simulink model "Copy_of_single_camera_q_dot"  (R2025b)
settings: Solver=FixedStepDiscrete  StartTime=0  StopTime=inf  FixedStep=Ts  RelTol=1e-3
InitFcn:
  | % 获取当前.slx模型所在文件夹
  | model_path = fileparts(which(gcs));
  | % 向上跳转、拼接目标函数所在文件夹（根据你的目录调整）
  | func_folder = fullfile(model_path,'..', 'config');
  | % 添加到搜索路径
  | addpath(func_folder);
  | % 执行初始化函数
  | init_single_camera_q_dot_tracking;
undefined symbols (not defined in the file or in its folder): camera_velocity_feedback_timeout_sec, controller_enable, cx, cy, data, data_SL_Info, depth_safe_max, depth_safe_min, depth_safety_gain, ekf_gate_threshold, enable_ekf_feedforward, enable_proportional, fx, fy, joint_acceleration_limit, joint_nominal_configuration, joint_position_max, joint_position_min, joint_soft_margin, joint_state_timeout_sec, joint_velocity_limit, k_ff, Kpx, Kpy, measurement_reset_timeout, nullspace_posture_gain, P0, Q_ekf, R_ekf, required_valid_frames, singularity_sigma_stop, singularity_sigma_warn, target_timeout_sec, task_velocity_filter_tau, Ts, visual_damping_max, visual_damping_min, visual_min_depth, Z_hat
libraries: ros2lib x4, robotmaniplib x2
(part 1 of 2)
Description:
  | Fixed-focus monocular XY target tracking. Outputs camera-frame [vx vy 0 0 0 0]; robot kinematics remain external.
settings Model: Creator=ASUS  LastModifiedBy=harry
settings DataIOCC: SignalLogging=off

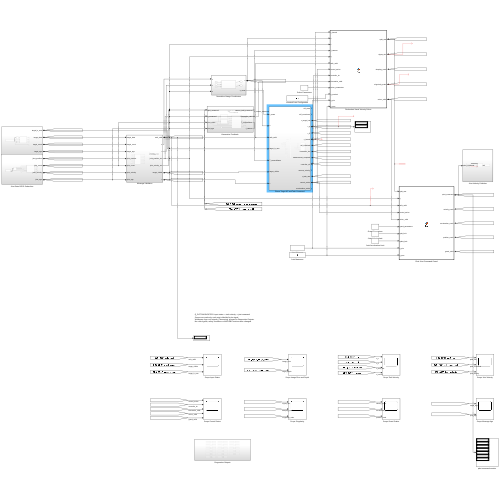
[thumbnail: Simulink's stored preview of the top-level diagram]
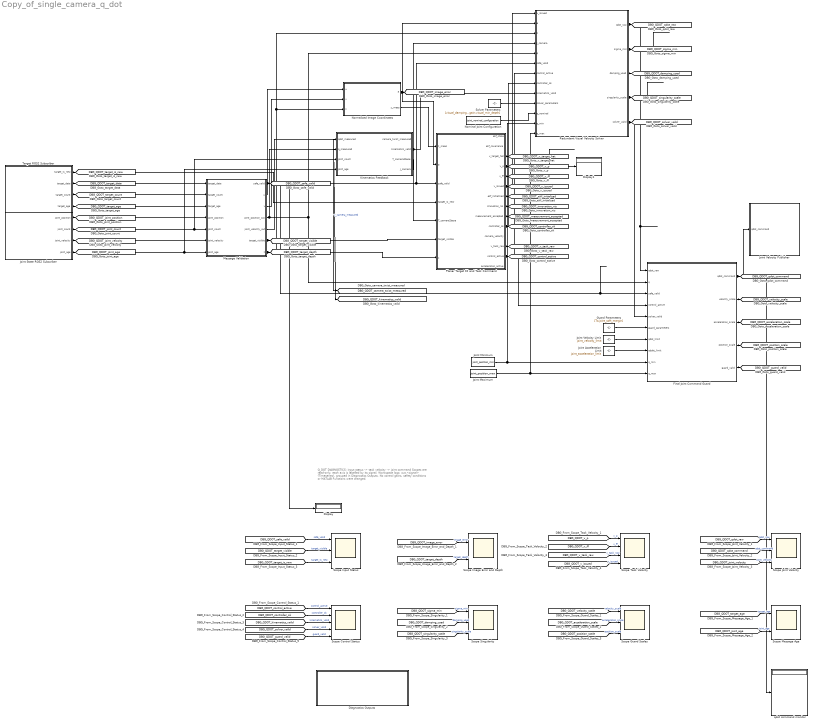
== system Copy_of_single_camera_q_dot ==
  note: Q_DOT DIAGNOSTICS: input status -> task velocity -> joint command
      | Scopes are read-only; each axis is labelled by its signal.
      | Workspace logs: out.<signal> (Timeseries), grouped in Diagnostics Outputs.
      | No control gains, safety conditions or MATLAB Functions were changed.
  Diagnostics Outputs : Subsystem
  Display : Display
  Display1 : Display
  Final Joint Command Guard : MATLAB Function  TreatAsAtomicUnit=on
  Guard Parameters : Constant  Value=[Ts;joint_soft_margin]
  Joint Acceleration Limit : Constant  Value=joint_acceleration_limit
  Joint Maximum : Constant  Value=joint_position_max
  Joint Minimum : Constant  Value=joint_position_min
  Joint State ROS2 Subscriber : Subsystem
  Joint Velocity Limit : Constant  Value=joint_velocity_limit
  Joint Velocity Publisher : Subsystem
  Kinematics Feedback : Subsystem
  Message Validation : Subsystem
  Nominal Joint Configuration : Constant  Value=joint_nominal_configuration
  Normalized Image Coordinates : Subsystem
  Planar Target KF and Task Command : Subsystem
  Redundant Visual Velocity Solver : MATLAB Function  TreatAsAtomicUnit=on
  Scope Control Status : Scope  NumInputPorts=5
      settings: TimeSpan=10  ActiveDisplayString=5  Title=guard_valid  ActiveDisplayYMinimum=-0.037001953201183713  ActiveDisplayYMaximum=0.0101088347899616  DataLoggingVariableName=ScopeData4
  Scope Guard Scales : Scope  NumInputPorts=3
      settings: TimeSpan=10  ActiveDisplayString=3  Title=position_scale  ActiveDisplayYMinimum=-12.068513318672558  ActiveDisplayYMaximum=6.6876450330275015  DataLoggingVariableName=ScopeData6
  Scope Image Error and Depth : Scope  NumInputPorts=2
      settings: TimeSpan=10  Title=target_depth  ActiveDisplayYMinimum=-1  ActiveDisplayYMaximum=1
  Scope Input Status : Scope  NumInputPorts=3
      settings: TimeSpan=10  ActiveDisplayString=3  Title=target_is_new  ActiveDisplayYMinimum=-1.6084422447956979  ActiveDisplayYMaximum=1.406793571934575  DataLoggingVariableName=ScopeData7
  Scope Joint Velocity : Scope  NumInputPorts=3
      settings: TimeSpan=10  ActiveDisplayString=3  Title=joint_velocity  ActiveDisplayYMinimum=-1.0517167509781138  ActiveDisplayYMaximum=1.0307773782957734  DataLoggingVariableName=ScopeData2
  Scope Message Age : Scope  NumInputPorts=2
      settings: TimeSpan=10  Title=joint_age  ActiveDisplayYMinimum=-1  ActiveDisplayYMaximum=1
  Scope Singularity : Scope  NumInputPorts=3
      settings: TimeSpan=10  ActiveDisplayString=3  Title=singularity_scale  ActiveDisplayYMinimum=-3.3735923675324466  ActiveDisplayYMaximum=2.902388236211491  DataLoggingVariableName=ScopeData5
  Scope Task Velocity : Scope  NumInputPorts=4
      settings: TimeSpan=10  ActiveDisplayString=4  Title=v_issued  ActiveDisplayYMinimum=-1  ActiveDisplayYMaximum=1  DataLoggingVariableName=ScopeData3
  Solver Parameters : Constant  Value=[visual_damping_min;visual_damping_max;singularity_sigma_stop;singularity_sigma_warn;nullspace_posture_gain;depth_safe_min;depth_safe_max;depth_safety_gain;visual_min_depth]
  Target ROS2 Subscriber : Subsystem
  qdot command monitor : Display
  tag scope: DBG_QDOT_acceleration_scale=global, DBG_QDOT_camera_twist_measured=global, DBG_QDOT_control_active=global, DBG_QDOT_controller_ok=global, DBG_QDOT_damping_used=global, DBG_QDOT_ekf_initialized=global, DBG_QDOT_guard_valid=global, DBG_QDOT_image_error=global, DBG_QDOT_innovation_nis=global, DBG_QDOT_joint_age=global, DBG_QDOT_joint_count=global, DBG_QDOT_joint_position=global, DBG_QDOT_joint_velocity=global, DBG_QDOT_kinematics_valid=global, DBG_QDOT_measurement_accepted=global, DBG_QDOT_position_scale=global, DBG_QDOT_qdot_command=global, DBG_QDOT_qdot_raw=global, DBG_QDOT_safe_valid=global, DBG_QDOT_sigma_min=global, DBG_QDOT_singularity_scale=global, DBG_QDOT_solver_valid=global, DBG_QDOT_target_age=global, DBG_QDOT_target_count=global, DBG_QDOT_target_data=global, DBG_QDOT_target_depth=global, DBG_QDOT_target_is_new=global, DBG_QDOT_target_visible=global, DBG_QDOT_v_ff=global, DBG_QDOT_v_issued=global, DBG_QDOT_v_p=global, DBG_QDOT_v_target_hat=global, DBG_QDOT_v_task_raw=global, DBG_QDOT_velocity_scale=global
  wires:
  Final Joint Command Guard/1(qdot_command) -> Joint Velocity Publisher/1(qdot_command), qdot command monitor/1, [DBG_QDOT_qdot_command]
  Message Validation/4(joint_position_out) -> Final Joint Command Guard/2(q), Redundant Visual Velocity Solver/5(q), Kinematics Feedback/2(q_measured)
  Kinematics Feedback/2(kinematics_valid) -> Redundant Visual Velocity Solver/9(kinematics_valid), [DBG_QDOT_kinematics_valid]
  Joint Velocity Limit/1 -> Final Joint Command Guard/7(qdot_limit)
  Message Validation/2(u) -> Normalized Image Coordinates/1(u)
  Target ROS2 Subscriber/3(target_count) -> Message Validation/2(target_count), [DBG_QDOT_target_count]
  Redundant Visual Velocity Solver/5(solver_valid) -> Final Joint Command Guard/5(solver_valid), [DBG_QDOT_solver_valid]
  Target ROS2 Subscriber/1(target_is_new) -> Planar Target KF and Task Command/4(target_is_new), [DBG_QDOT_target_is_new]
  Planar Target KF and Task Command/10(controller_ok) -> Redundant Visual Velocity Solver/8(controller_ok), [DBG_QDOT_controller_ok]
  Message Validation/5(joint_velocity_out) -> Kinematics Feedback/1(qdot_measured)
  Message Validation/7(z) -> Redundant Visual Velocity Solver/3(z), Normalized Image Coordinates/3(z), Planar Target KF and Task Command/7(z), [DBG_QDOT_target_depth]
  Joint Acceleration Limit/1 -> Final Joint Command Guard/8(qddot_limit)
  Joint State ROS2 Subscriber/4(joint_age) -> Kinematics Feedback/4(joint_age), Message Validation/7(joint_age), [DBG_QDOT_joint_age]
  Joint State ROS2 Subscriber/3(joint_velocity) -> Message Validation/6(joint_velocity), [DBG_QDOT_joint_velocity]
  Message Validation/6(target_visible) -> Planar Target KF and Task Command/6(target_visible), [DBG_QDOT_target_visible]
  Kinematics Feedback/4(J_camera) -> Redundant Visual Velocity Solver/4(J_camera)
  Redundant Visual Velocity Solver/1(qdot_raw) -> [DBG_QDOT_qdot_raw], Final Joint Command Guard/1(qdot_raw)
  Message Validation/1(safe_valid) -> Final Joint Command Guard/3(safe_valid), Redundant Visual Velocity Solver/6(safe_valid), Planar Target KF and Task Command/3(safe_valid), Display/1, [DBG_QDOT_safe_valid]
  Message Validation/3(v) -> Normalized Image Coordinates/2(v)
  Planar Target KF and Task Command/13(control_active) -> Redundant Visual Velocity Solver/7(control_active), Final Joint Command Guard/4(control_active), [DBG_QDOT_control_active]
  Joint State ROS2 Subscriber/1(joint_position) -> Message Validation/4(joint_position), [DBG_QDOT_joint_position]
  Guard Parameters/1 -> Final Joint Command Guard/6(guard_parameters)
  Joint State ROS2 Subscriber/2(joint_count) -> Kinematics Feedback/3(joint_count), Message Validation/5(joint_count), [DBG_QDOT_joint_count]
  Normalized Image Coordinates/1(e) -> Planar Target KF and Task Command/2(e), Redundant Visual Velocity Solver/2(e), [DBG_QDOT_image_error]
  Target ROS2 Subscriber/2(target_data) -> Message Validation/1(target_data), [DBG_QDOT_target_data]
  Normalized Image Coordinates/2(z_meas) -> Planar Target KF and Task Command/1(z_meas)
  Kinematics Feedback/3(T_camera2base) -> Planar Target KF and Task Command/5(T_camera2base)
  Solver Parameters/1 -> Redundant Visual Velocity Solver/10(solver_parameters)
  Nominal Joint Configuration/1 -> Redundant Visual Velocity Solver/11(q_nominal)
  Joint Minimum/1 -> Redundant Visual Velocity Solver/12(q_min), Final Joint Command Guard/9(q_min)
  Joint Maximum/1 -> Final Joint Command Guard/10(q_max), Redundant Visual Velocity Solver/13(q_max)
  Target ROS2 Subscriber/4(target_age) -> Message Validation/3(target_age), [DBG_QDOT_target_age]
  Planar Target KF and Task Command/4(v_p) -> Display1/1, [DBG_QDOT_v_p]
  Planar Target KF and Task Command/6(v_issued) -> Redundant Visual Velocity Solver/1(v_issued), [DBG_QDOT_v_issued]
  Redundant Visual Velocity Solver/2(sigma_min) -> [DBG_QDOT_sigma_min]
  Redundant Visual Velocity Solver/4(singularity_scale) -> [DBG_QDOT_singularity_scale]
  Kinematics Feedback/1(camera_twist_measured) -> [DBG_QDOT_camera_twist_measured]  "v_camera_measured"
  Planar Target KF and Task Command/3(v_target_hat) -> [DBG_QDOT_v_target_hat]
  Planar Target KF and Task Command/5(v_ff) -> [DBG_QDOT_v_ff]
  Planar Target KF and Task Command/7(ekf_initialized) -> [DBG_QDOT_ekf_initialized]
  Planar Target KF and Task Command/8(innovation_nis) -> [DBG_QDOT_innovation_nis]
  Planar Target KF and Task Command/9(measurement_accepted) -> [DBG_QDOT_measurement_accepted]
  Planar Target KF and Task Command/12(v_task_raw) -> [DBG_QDOT_v_task_raw]
  Redundant Visual Velocity Solver/3(damping_used) -> [DBG_QDOT_damping_used]
  Final Joint Command Guard/2(velocity_scale) -> [DBG_QDOT_velocity_scale]
  Final Joint Command Guard/3(acceleration_scale) -> [DBG_QDOT_acceleration_scale]
  Final Joint Command Guard/4(position_scale) -> [DBG_QDOT_position_scale]
  Final Joint Command Guard/5(guard_valid) -> [DBG_QDOT_guard_valid]
  [DBG_QDOT_safe_valid] -> Scope Input Status/1  "safe_valid"
  [DBG_QDOT_target_visible] -> Scope Input Status/2  "target_visible"
  [DBG_QDOT_target_is_new] -> Scope Input Status/3  "target_is_new"
  [DBG_QDOT_image_error] -> Scope Image Error and Depth/1  "image_error"
  [DBG_QDOT_target_depth] -> Scope Image Error and Depth/2  "target_depth"
  [DBG_QDOT_v_p] -> Scope Task Velocity/1  "v_p"
  [DBG_QDOT_v_ff] -> Scope Task Velocity/2  "v_ff"
  [DBG_QDOT_v_task_raw] -> Scope Task Velocity/3  "v_task_raw"
  [DBG_QDOT_v_issued] -> Scope Task Velocity/4  "v_issued"
  [DBG_QDOT_qdot_raw] -> Scope Joint Velocity/1  "qdot_raw"
  [DBG_QDOT_qdot_command] -> Scope Joint Velocity/2  "qdot_command"
  [DBG_QDOT_joint_velocity] -> Scope Joint Velocity/3  "joint_velocity"
  [DBG_QDOT_control_active] -> Scope Control Status/1  "control_active"
  [DBG_QDOT_controller_ok] -> Scope Control Status/2  "controller_ok"
  [DBG_QDOT_kinematics_valid] -> Scope Control Status/3  "kinematics_valid"
  [DBG_QDOT_solver_valid] -> Scope Control Status/4  "solver_valid"
  [DBG_QDOT_guard_valid] -> Scope Control Status/5  "guard_valid"
  [DBG_QDOT_sigma_min] -> Scope Singularity/1  "sigma_min"
  [DBG_QDOT_damping_used] -> Scope Singularity/2  "damping_used"
  [DBG_QDOT_singularity_scale] -> Scope Singularity/3  "singularity_scale"
  [DBG_QDOT_velocity_scale] -> Scope Guard Scales/1  "velocity_scale"
  [DBG_QDOT_acceleration_scale] -> Scope Guard Scales/2  "acceleration_scale"
  [DBG_QDOT_position_scale] -> Scope Guard Scales/3  "position_scale"
  [DBG_QDOT_target_age] -> Scope Message Age/1  "target_age"
  [DBG_QDOT_joint_age] -> Scope Message Age/2  "joint_age"

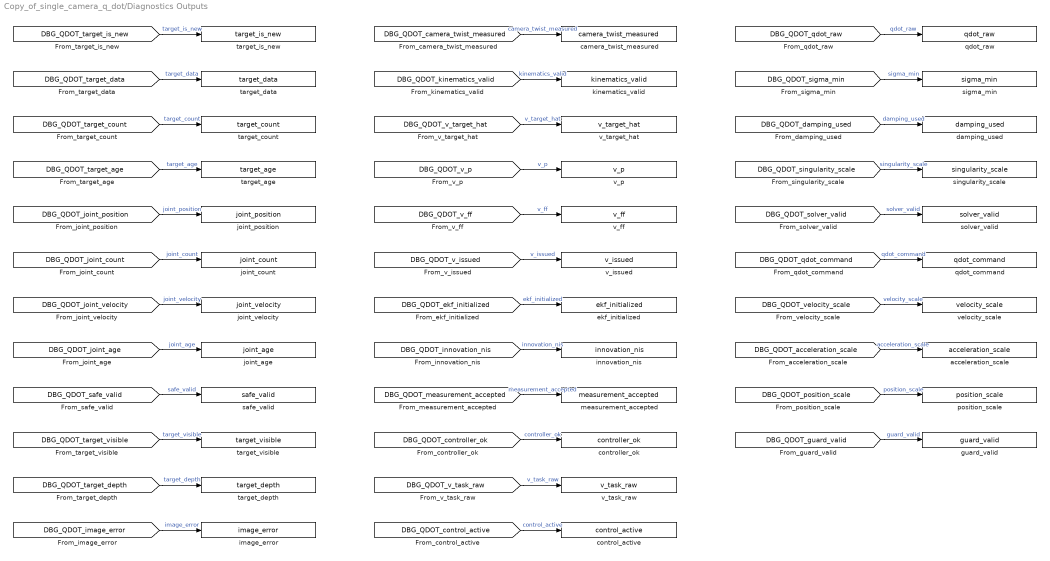
== system Copy_of_single_camera_q_dot/Diagnostics Outputs ==
  acceleration_scale : ToWorkspace  VariableName=acceleration_scale  SaveFormat=Timeseries  SampleTime=-1
  camera_twist_measured : ToWorkspace  VariableName=camera_twist_measured  SaveFormat=Timeseries  SampleTime=-1
  control_active : ToWorkspace  VariableName=control_active  SaveFormat=Timeseries  SampleTime=-1
  controller_ok : ToWorkspace  VariableName=controller_ok  SaveFormat=Timeseries  SampleTime=-1
  damping_used : ToWorkspace  VariableName=damping_used  SaveFormat=Timeseries  SampleTime=-1
  ekf_initialized : ToWorkspace  VariableName=ekf_initialized  SaveFormat=Timeseries  SampleTime=-1
  guard_valid : ToWorkspace  VariableName=guard_valid  SaveFormat=Timeseries  SampleTime=-1
  image_error : ToWorkspace  VariableName=image_error  SaveFormat=Timeseries  SampleTime=-1
  innovation_nis : ToWorkspace  VariableName=innovation_nis  SaveFormat=Timeseries  SampleTime=-1
  joint_age : ToWorkspace  VariableName=joint_age  SaveFormat=Timeseries  SampleTime=-1
  joint_count : ToWorkspace  VariableName=joint_count  SaveFormat=Timeseries  SampleTime=-1
  joint_position : ToWorkspace  VariableName=joint_position  SaveFormat=Timeseries  SampleTime=-1
  joint_velocity : ToWorkspace  VariableName=joint_velocity  SaveFormat=Timeseries  SampleTime=-1
  kinematics_valid : ToWorkspace  VariableName=kinematics_valid  SaveFormat=Timeseries  SampleTime=-1
  measurement_accepted : ToWorkspace  VariableName=measurement_accepted  SaveFormat=Timeseries  SampleTime=-1
  position_scale : ToWorkspace  VariableName=position_scale  SaveFormat=Timeseries  SampleTime=-1
  qdot_command : ToWorkspace  VariableName=qdot_command  SaveFormat=Timeseries  SampleTime=-1
  qdot_raw : ToWorkspace  VariableName=qdot_raw  SaveFormat=Timeseries  SampleTime=-1
  safe_valid : ToWorkspace  VariableName=safe_valid  SaveFormat=Timeseries  SampleTime=-1
  sigma_min : ToWorkspace  VariableName=sigma_min  SaveFormat=Timeseries  SampleTime=-1
  singularity_scale : ToWorkspace  VariableName=singularity_scale  SaveFormat=Timeseries  SampleTime=-1
  solver_valid : ToWorkspace  VariableName=solver_valid  SaveFormat=Timeseries  SampleTime=-1
  target_age : ToWorkspace  VariableName=target_age  SaveFormat=Timeseries  SampleTime=-1
  target_count : ToWorkspace  VariableName=target_count  SaveFormat=Timeseries  SampleTime=-1
  target_data : ToWorkspace  VariableName=target_data  SaveFormat=Timeseries  SampleTime=-1
  target_depth : ToWorkspace  VariableName=target_depth  SaveFormat=Timeseries  SampleTime=-1
  target_is_new : ToWorkspace  VariableName=target_is_new  SaveFormat=Timeseries  SampleTime=-1
  target_visible : ToWorkspace  VariableName=target_visible  SaveFormat=Timeseries  SampleTime=-1
  v_ff : ToWorkspace  VariableName=v_ff  SaveFormat=Timeseries  SampleTime=-1
  v_issued : ToWorkspace  VariableName=v_issued  SaveFormat=Timeseries  SampleTime=-1
  v_p : ToWorkspace  VariableName=v_p  SaveFormat=Timeseries  SampleTime=-1
  v_target_hat : ToWorkspace  VariableName=v_target_hat  SaveFormat=Timeseries  SampleTime=-1
  v_task_raw : ToWorkspace  VariableName=v_task_raw  SaveFormat=Timeseries  SampleTime=-1
  velocity_scale : ToWorkspace  VariableName=velocity_scale  SaveFormat=Timeseries  SampleTime=-1
  wires:
  [DBG_QDOT_target_is_new] -> target_is_new/1  "target_is_new"
  [DBG_QDOT_target_data] -> target_data/1  "target_data"
  [DBG_QDOT_target_count] -> target_count/1  "target_count"
  [DBG_QDOT_target_age] -> target_age/1  "target_age"
  [DBG_QDOT_joint_position] -> joint_position/1  "joint_position"
  [DBG_QDOT_joint_count] -> joint_count/1  "joint_count"
  [DBG_QDOT_joint_velocity] -> joint_velocity/1  "joint_velocity"
  [DBG_QDOT_joint_age] -> joint_age/1  "joint_age"
  [DBG_QDOT_safe_valid] -> safe_valid/1  "safe_valid"
  [DBG_QDOT_target_visible] -> target_visible/1  "target_visible"
  [DBG_QDOT_target_depth] -> target_depth/1  "target_depth"
  [DBG_QDOT_image_error] -> image_error/1  "image_error"
  [DBG_QDOT_camera_twist_measured] -> camera_twist_measured/1  "camera_twist_measured"
  [DBG_QDOT_kinematics_valid] -> kinematics_valid/1  "kinematics_valid"
  [DBG_QDOT_v_target_hat] -> v_target_hat/1  "v_target_hat"
  [DBG_QDOT_v_p] -> v_p/1  "v_p"
  [DBG_QDOT_v_ff] -> v_ff/1  "v_ff"
  [DBG_QDOT_v_issued] -> v_issued/1  "v_issued"
  [DBG_QDOT_ekf_initialized] -> ekf_initialized/1  "ekf_initialized"
  [DBG_QDOT_innovation_nis] -> innovation_nis/1  "innovation_nis"
  [DBG_QDOT_measurement_accepted] -> measurement_accepted/1  "measurement_accepted"
  [DBG_QDOT_controller_ok] -> controller_ok/1  "controller_ok"
  [DBG_QDOT_v_task_raw] -> v_task_raw/1  "v_task_raw"
  [DBG_QDOT_control_active] -> control_active/1  "control_active"
  [DBG_QDOT_qdot_raw] -> qdot_raw/1  "qdot_raw"
  [DBG_QDOT_sigma_min] -> sigma_min/1  "sigma_min"
  [DBG_QDOT_damping_used] -> damping_used/1  "damping_used"
  [DBG_QDOT_singularity_scale] -> singularity_scale/1  "singularity_scale"
  [DBG_QDOT_solver_valid] -> solver_valid/1  "solver_valid"
  [DBG_QDOT_qdot_command] -> qdot_command/1  "qdot_command"
  [DBG_QDOT_velocity_scale] -> velocity_scale/1  "velocity_scale"
  [DBG_QDOT_acceleration_scale] -> acceleration_scale/1  "acceleration_scale"
  [DBG_QDOT_position_scale] -> position_scale/1  "position_scale"
  [DBG_QDOT_guard_valid] -> guard_valid/1  "guard_valid"

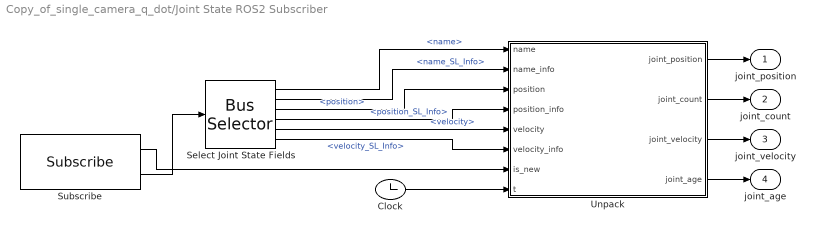
== system Copy_of_single_camera_q_dot/Joint State ROS2 Subscriber ==
  Clock : Clock
  Select Joint State Fields : BusSelector  OutputSignals=name,name_SL_Info,position,position_SL_Info,velocity,velocity_SL_Info
  Subscribe : ros2lib/Subscribe  topicSource=Select from ROS network  topic=/franka/joint_states  messageType=sensor_msgs/JointState  sampleTime=Ts  QOSHistory=Keep last  QOSDepth=1  QOSReliability=Best effort  QOSDurability=Volatile  QOSDeadline=Inf  QOSLifespan=Inf  QOSLiveliness=Automatic  QOSLeaseDuration=Inf  QOSAvoidROSNamespaceConventions=off
  Unpack : MATLAB Function  TreatAsAtomicUnit=on
  joint_position : Outport
  joint_count : Outport  Port=2
  joint_velocity : Outport  Port=3
  joint_age : Outport  Port=4
  wires:
  Unpack/1(joint_position) -> joint_position/1
  Unpack/2(joint_count) -> joint_count/1
  Unpack/3(joint_velocity) -> joint_velocity/1
  Unpack/4(joint_age) -> joint_age/1
  Subscribe/2 -> Select Joint State Fields/1
  Select Joint State Fields/1 -> Unpack/1(name)  "<name>"
  Select Joint State Fields/2 -> Unpack/2(name_info)  "<name_SL_Info>"
  Select Joint State Fields/3 -> Unpack/3(position)  "<position>"
  Select Joint State Fields/4 -> Unpack/4(position_info)  "<position_SL_Info>"
  Select Joint State Fields/5 -> Unpack/5(velocity)  "<velocity>"
  Select Joint State Fields/6 -> Unpack/6(velocity_info)  "<velocity_SL_Info>"
  Subscribe/1 -> Unpack/7(is_new)
  Clock/1 -> Unpack/8(t)

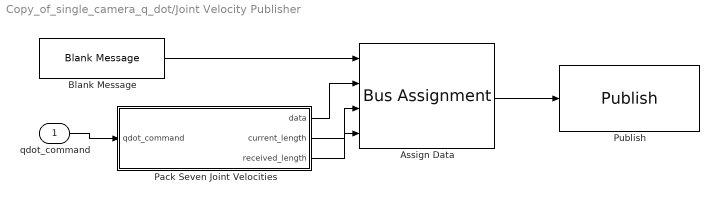
== system Copy_of_single_camera_q_dot/Joint Velocity Publisher ==
  qdot_command : Inport
  Assign Data : BusAssignment  AssignedSignals=data,data_SL_Info.CurrentLength,data_SL_Info.ReceivedLength
  Blank Message : ros2lib/Blank Message  messageClass=Message  entityType=std_msgs/Float64MultiArray  messageType=std_msgs/Float64MultiArray  SampleTime=Ts
  Pack Seven Joint Velocities : MATLAB Function  TreatAsAtomicUnit=on
  Publish : ros2lib/Publish  topicSource=Select from ROS network  topic=/joint_velocity_example_controller/commands  messageType=std_msgs/Float64MultiArray  QOSHistory=Keep last  QOSDepth=1  QOSReliability=Reliable  QOSDurability=Volatile  QOSDeadline=Inf  QOSLifespan=Inf  QOSLiveliness=Automatic  QOSLeaseDuration=Inf  QOSAvoidROSNamespaceConventions=off
  wires:
  ? -> ?
  qdot_command/1 -> Pack Seven Joint Velocities/1(qdot_command)
  Blank Message/1 -> Assign Data/1
  Pack Seven Joint Velocities/1(data) -> Assign Data/2
  Pack Seven Joint Velocities/2(current_length) -> Assign Data/3
  Pack Seven Joint Velocities/3(received_length) -> Assign Data/4
  Assign Data/1 -> Publish/1

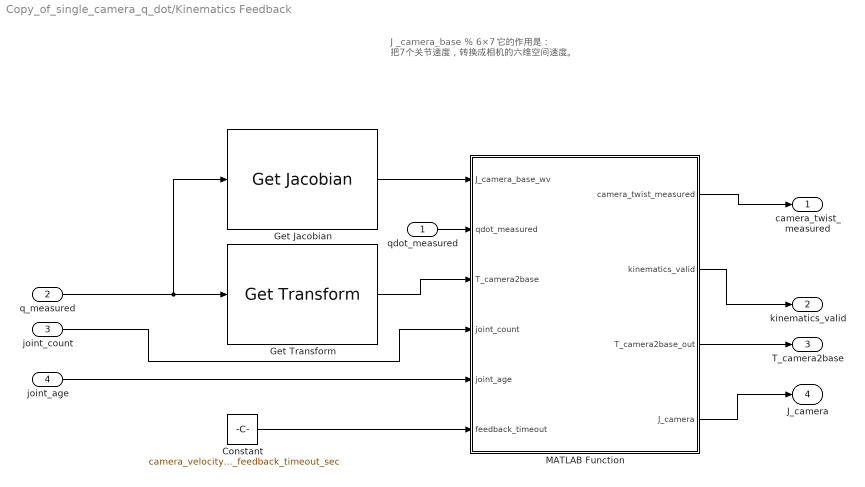
== system Copy_of_single_camera_q_dot/Kinematics Feedback ==
  note: J _camera_base % 6×7
      | 它的作用是：
      | 把7个关节速度，转换成相机的六维空间速度。
  qdot_measured : Inport
  q_measured : Inport  Port=2
  joint_count : Inport  Port=3
  joint_age : Inport  Port=4
  Constant : Constant  Value=camera_velocity_feedback_timeout_sec
  Get Jacobian : robotmaniplib/Get Jacobian  RigidBodyTree=fr3_camera_robot  EndEffector=camera_link  SimulateUsing=Interpreted execution
  Get Transform : robotmaniplib/Get Transform  RigidBodyTree=fr3_camera_robot  SourceBody=camera_link  TargetBody=base  SimulateUsing=Interpreted execution
  MATLAB Function : MATLAB Function  TreatAsAtomicUnit=on
  camera_twist_measured : Outport
  kinematics_valid : Outport  Port=2
  T_camera2base : Outport  Port=3
  J_camera : Outport  Port=4
  wires:
  q_measured/1 -> Get Jacobian/1, Get Transform/1
  qdot_measured/1 -> MATLAB Function/2(qdot_measured)
  Get Jacobian/1 -> MATLAB Function/1(J_camera_base_wv)
  Get Transform/1 -> MATLAB Function/3(T_camera2base)
  joint_count/1 -> MATLAB Function/4(joint_count)
  joint_age/1 -> MATLAB Function/5(joint_age)
  Constant/1 -> MATLAB Function/6(feedback_timeout)
  MATLAB Function/1(camera_twist_measured) -> camera_twist_measured/1
  MATLAB Function/2(kinematics_valid) -> kinematics_valid/1
  MATLAB Function/3(T_camera2base_out) -> T_camera2base/1
  MATLAB Function/4(J_camera) -> J_camera/1

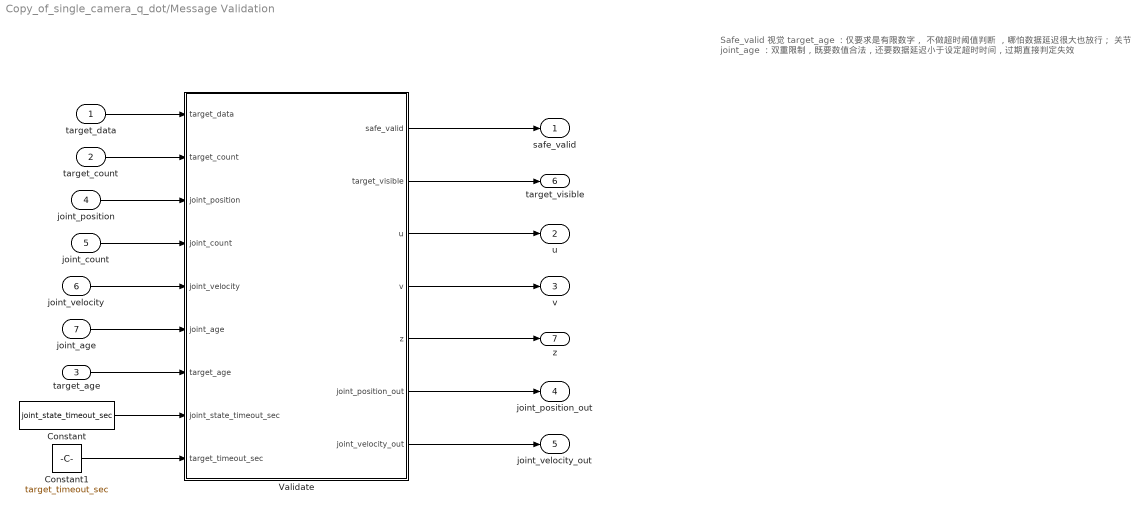
== system Copy_of_single_camera_q_dot/Message Validation ==
  note: Safe_valid
      | 视觉 target_age ：仅要求是有限数字， 不做超时阈值判断 ，哪怕数据延迟很大也放行；
      | 关节 joint_age ：双重限制，既要数值合法，还要数据延迟小于设定超时时间，过期直接判定失效
  target_data : Inport
  target_count : Inport  Port=2
  target_age : Inport  Port=3
  joint_position : Inport  Port=4
  joint_count : Inport  Port=5
  joint_velocity : Inport  Port=6
  joint_age : Inport  Port=7
  Constant : Constant  Value=joint_state_timeout_sec
  Constant1 : Constant  Value=target_timeout_sec
  Validate : MATLAB Function  TreatAsAtomicUnit=on
  safe_valid : Outport
  u : Outport  Port=2
  v : Outport  Port=3
  joint_position_out : Outport  Port=4
  joint_velocity_out : Outport  Port=5
  target_visible : Outport  Port=6
  z : Outport  Port=7
  wires:
  Validate/1(safe_valid) -> safe_valid/1
  Validate/3(u) -> u/1
  Validate/4(v) -> v/1
  Validate/6(joint_position_out) -> joint_position_out/1
  Validate/7(joint_velocity_out) -> joint_velocity_out/1
  target_data/1 -> Validate/1(target_data)
  target_count/1 -> Validate/2(target_count)
  Validate/2(target_visible) -> target_visible/1
  joint_position/1 -> Validate/3(joint_position)
  joint_count/1 -> Validate/4(joint_count)
  joint_velocity/1 -> Validate/5(joint_velocity)
  joint_age/1 -> Validate/6(joint_age)
  Constant/1 -> Validate/8(joint_state_timeout_sec)
  Validate/5(z) -> z/1
  target_age/1 -> Validate/7(target_age)
  Constant1/1 -> Validate/9(target_timeout_sec)

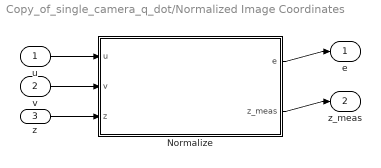
== system Copy_of_single_camera_q_dot/Normalized Image Coordinates ==
  u : Inport
  v : Inport  Port=2
  z : Inport  Port=3
  Normalize : MATLAB Function  TreatAsAtomicUnit=on
  e : Outport
  z_meas : Outport  Port=2
  wires:
  u/1 -> Normalize/1(u)
  v/1 -> Normalize/2(v)
  Normalize/1(e) -> e/1
  Normalize/2(z_meas) -> z_meas/1
  z/1 -> Normalize/3(z)

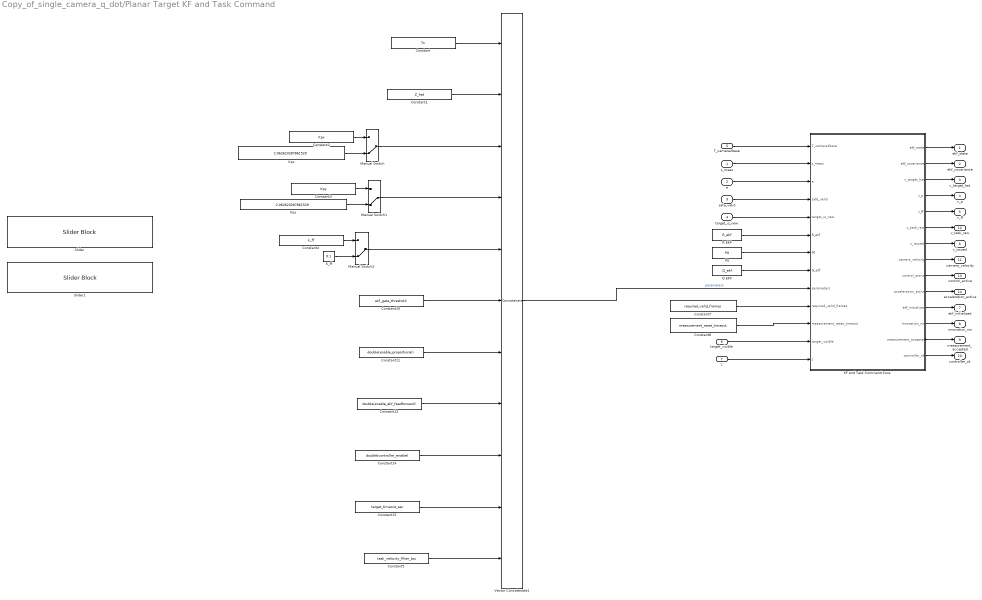
== system Copy_of_single_camera_q_dot/Planar Target KF and Task Command ==
  z_meas : Inport
  e : Inport  Port=2
  safe_valid : Inport  Port=3
  target_is_new : Inport  Port=4
  T_camera2base : Inport  Port=5
  target_visible : Inport  Port=6
  z : Inport  Port=7
  Constant : Constant  Value=Ts
  Constant1 : Constant  Value=Z_hat
  Constant10 : Constant  Value=ekf_gate_threshold
  Constant11 : Constant  Value=double(enable_proportional)
  Constant12 : Constant  Value=double(enable_ekf_feedforward)
  Constant14 : Constant  Value=double(controller_enable)
  Constant15 : Constant  Value=target_timeout_sec
  Constant2 : Constant  Value=Kpx
  Constant3 : Constant  Value=Kpy
  Constant4 : Constant  Value=k_ff
  Constant5 : Constant  Value=task_velocity_filter_tau
  Constant7 : Constant  Value=required_valid_frames
  Constant8 : Constant  Value=measurement_reset_timeout
  KF and Task Command Core : MATLAB Function  TreatAsAtomicUnit=on
  K_ff : Constant  Value=0.1
  Kpx : Constant  Value=2.062623287861529
  Kpy : Constant  Value=2.062623287861529
  Manual Switch : ManualSwitch  CurrentSetting=0
  Manual Switch1 : ManualSwitch  CurrentSetting=0
  Manual Switch2 : ManualSwitch  CurrentSetting=0
  P0 : Constant  Value=P0
  Q EKF : Constant  Value=Q_ekf
  R EKF : Constant  Value=R_ekf
  Slider : SliderBlock  ScaleMax=10
  Slider1 : SliderBlock  ScaleMax=10
  Vector Concatenate1 : Concatenate  NumInputs=11
  ekf_state : Outport
  ekf_covariance : Outport  Port=2
  v_target_hat : Outport  Port=3
  v_p : Outport  Port=4
  v_ff : Outport  Port=5
  v_issued : Outport  Port=6
  ekf_initialized : Outport  Port=7
  innovation_nis : Outport  Port=8
  measurement_accepted : Outport  Port=9
  controller_ok : Outport  Port=10
  camera_velocity : Outport  Port=11
  v_task_raw : Outport  Port=12
  control_active : Outport  Port=13
  acceleration_active : Outport  Port=14
  wires:
  KF and Task Command Core/1(ekf_state) -> ekf_state/1
  KF and Task Command Core/2(ekf_covariance) -> ekf_covariance/1
  KF and Task Command Core/3(v_target_hat) -> v_target_hat/1
  KF and Task Command Core/4(v_p) -> v_p/1
  KF and Task Command Core/5(v_ff) -> v_ff/1
  KF and Task Command Core/7(v_issued) -> v_issued/1
  KF and Task Command Core/8(camera_velocity) -> camera_velocity/1
  KF and Task Command Core/11(ekf_initialized) -> ekf_initialized/1
  KF and Task Command Core/12(innovation_nis) -> innovation_nis/1
  KF and Task Command Core/13(measurement_accepted) -> measurement_accepted/1
  KF and Task Command Core/14(controller_ok) -> controller_ok/1
  z_meas/1 -> KF and Task Command Core/2(z_meas)
  e/1 -> KF and Task Command Core/3(e)
  safe_valid/1 -> KF and Task Command Core/4(safe_valid)
  target_is_new/1 -> KF and Task Command Core/5(target_is_new)
  Vector Concatenate1/1 -> KF and Task Command Core/9(parameters)  "parameters"
  P0/1 -> KF and Task Command Core/7(P0)
  Q EKF/1 -> KF and Task Command Core/8(Q_ekf)
  R EKF/1 -> KF and Task Command Core/6(R_ekf)
  Constant/1 -> Vector Concatenate1/1
  Constant1/1 -> Vector Concatenate1/2
  Constant10/1 -> Vector Concatenate1/6
  Constant11/1 -> Vector Concatenate1/7
  Constant12/1 -> Vector Concatenate1/8
  Constant14/1 -> Vector Concatenate1/9
  Constant15/1 -> Vector Concatenate1/10
  T_camera2base/1 -> KF and Task Command Core/1(T_camera2base)
  Constant2/1 -> Manual Switch/1
  Manual Switch/1 -> Vector Concatenate1/3
  Kpx/1 -> Manual Switch/2
  Kpy/1 -> Manual Switch1/2
  Constant3/1 -> Manual Switch1/1
  Manual Switch1/1 -> Vector Concatenate1/4
  Constant4/1 -> Manual Switch2/1
  Manual Switch2/1 -> Vector Concatenate1/5
  K_ff/1 -> Manual Switch2/2
  KF and Task Command Core/6(v_task_raw) -> v_task_raw/1
  KF and Task Command Core/10(acceleration_active) -> acceleration_active/1
  KF and Task Command Core/9(control_active) -> control_active/1
  ? -> ?
  ? -> ?
  Constant7/1 -> KF and Task Command Core/10(required_valid_frames)
  Constant8/1 -> KF and Task Command Core/11(measurement_reset_timeout)
  target_visible/1 -> KF and Task Command Core/12(target_visible)
  z/1 -> KF and Task Command Core/13(z)
  Constant5/1 -> Vector Concatenate1/11

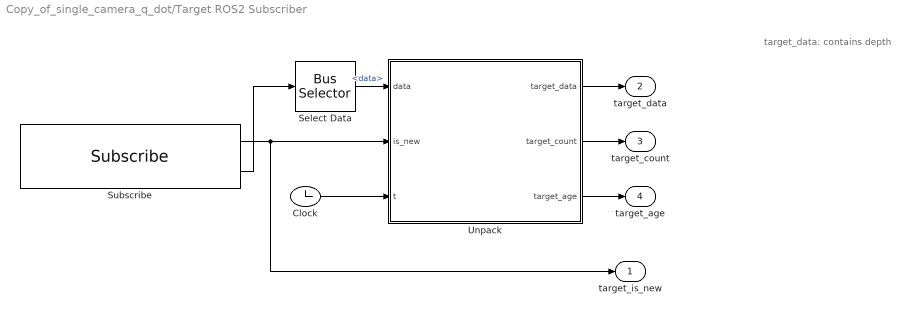
== system Copy_of_single_camera_q_dot/Target ROS2 Subscriber ==
  note: target_data: contains depth
  Clock : Clock
  Select Data : BusSelector  OutputSignals=data
  Subscribe : ros2lib/Subscribe  topicSource=Select from ROS network  topic=/apriltag_detector/target_position  messageType=std_msgs/Float64MultiArray  sampleTime=Ts  QOSHistory=Keep last  QOSDepth=1  QOSReliability=Best effort  QOSDurability=Volatile  QOSDeadline=Inf  QOSLifespan=Inf  QOSLiveliness=Automatic  QOSLeaseDuration=Inf  QOSAvoidROSNamespaceConventions=off
  Unpack : MATLAB Function  TreatAsAtomicUnit=on
  target_is_new : Outport
  target_data : Outport  Port=2
  target_count : Outport  Port=3
  target_age : Outport  Port=4
  wires:
  Unpack/1(target_data) -> target_data/1
  Unpack/2(target_count) -> target_count/1
  Unpack/3(target_age) -> target_age/1
  Select Data/1 -> Unpack/1(data)  "<data>"
  Clock/1 -> Unpack/3(t)
  Subscribe/2 -> Select Data/1
  Subscribe/1 -> target_is_new/1, Unpack/2(is_new)

== matlab function Copy_of_single_camera_q_dot/Normalized Image Coordinates/Normalize ==
  data: u input size=1; e output size=[2 1]; v input size=1; z_meas output size=[2 1]; fx parameter size=1; fy parameter size=1; cx parameter size=1; cy parameter size=1; z input
function [e,z_meas] = fcn(u,v, fx, fy, cx, cy,z)
%#codegen
ex=(u-cx)/fx; ey=(v-cy)/fy;
e=[ex;ey]; z_meas=z*e;
end

== matlab function Copy_of_single_camera_q_dot/Planar Target KF and Task Command/KF and Task Command Core ==
  data: T_camera2base input; z_meas input size=[2 1]; ekf_state output size=[4 1]; e input size=[2 1]; safe_valid input size=1; target_is_new input; R_ekf input size=[2 2]; P0 input size=[4 4]; Q_ekf input size=[4 4]; parameters input size=[11 1]; ekf_covariance output size=[4 4]; v_target_hat output size=[2 1]; v_p output size=[2 1]; v_ff output size=[2 1]; v_task_raw output; v_issued output size=[2 1]; camera_velocity output size=[6 1]; control_active output; acceleration_active output; ekf_initialized output size=1; innovation_nis output size=1; measurement_accepted output size=1; controller_ok output size=1; required_valid_frames input; measurement_reset_timeout input; target_visible input; z input
function [ekf_state,ekf_covariance,v_target_hat,v_p,v_ff,v_task_raw,v_issued,camera_velocity,control_active,acceleration_active,ekf_initialized,innovation_nis,measurement_accepted,controller_ok] = fcn( ...
T_camera2base,z_meas,e,safe_valid,target_is_new,R_ekf,P0,Q_ekf,parameters,required_valid_frames,measurement_reset_timeout,target_visible,z)
%#codegen
% 四状态匀速 KF：[X_B;Y_B;Vx_B;Vy_B]。
% 原消息、目标、P/FF 和总控制使能关系保持不变。
% v_task_raw 是未滤波、未限幅的二维相机平移速度请求。
% v_issued 是经过任务空间低通后的二维速度指令。

persistent x_hat P e_hold z_hold time_since_accepted initialized
persistent valid_streak ekf_ready time_since_visible target_tracking_active
persistent v_issued_hold

if isempty(initialized)
x_hat=zeros(4,1); P=P0; e_hold=zeros(2,1); z_hold=0.0;
time_since_accepted=0.0; initialized=false;
valid_streak=0.0; ekf_ready=false;
time_since_visible=inf; target_tracking_active=false;
v_issued_hold=zeros(2,1);
end

ekf_state=x_hat; ekf_covariance=P; v_target_hat=zeros(2,1);
v_p=zeros(2,1); v_ff=zeros(2,1); v_task_raw=zeros(2,1);
v_issued=zeros(2,1); camera_velocity=zeros(6,1);
control_active=false; acceleration_active=false;
ekf_initialized=initialized && ekf_ready; innovation_nis=NaN;
measurement_accepted=false; controller_ok=false;

if numel(parameters)<11
x_hat=zeros(4,1); P=P0; e_hold=zeros(2,1); z_hold=0.0;
time_since_accepted=0.0; initialized=false; valid_streak=0.0;
ekf_ready=false; time_since_visible=inf; target_tracking_active=false;
v_issued_hold=zeros(2,1);
ekf_state=x_hat; ekf_covariance=P; ekf_initialized=false; return;
end

Ts=parameters(1); Z_hat=parameters(2); Kpx=parameters(3); Kpy=parameters(4);
k_ff=parameters(5); gate=parameters(6);
enable_p=parameters(7)>0.5; enable_ff=parameters(8)>0.5;
controller_enable=parameters(9)>0.5;
target_lost_timeout=parameters(10);
task_velocity_filter_tau=parameters(11);

if target_lost_timeout<=0.0, target_lost_timeout=0.10; end

safe_valid=safe_valid>0.5; target_visible=target_visible>0.5;
target_is_new=target_is_new>0.5;
required_valid_frames=max(1.0,floor(required_valid_frames));

parameter_ok=all(isfinite(parameters(1:11))) && ...
isfinite(required_valid_frames) && isfinite(measurement_reset_timeout) && ...
Ts>0.0 && Z_hat>0.0 && gate>0.0 && task_velocity_filter_tau>=0.0 && ...
measurement_reset_timeout>=Ts && target_lost_timeout>=Ts && ...
isequal(size(R_ekf),[2 2]) && isequal(size(P0),[4 4]) && ...
isequal(size(Q_ekf),[4 4]) && all(isfinite(R_ekf(:))) && ...
all(isfinite(P0(:))) && all(isfinite(Q_ekf(:)));

if ~parameter_ok
x_hat=zeros(4,1); P=P0; e_hold=zeros(2,1); z_hold=0.0;
time_since_accepted=0.0; initialized=false; valid_streak=0.0;
ekf_ready=false; time_since_visible=inf; target_tracking_active=false;
v_issued_hold=zeros(2,1);
ekf_state=x_hat; ekf_covariance=P; ekf_initialized=false; return;
end

if ~(isfinite(z_hold) && z_hold>0.0)
z_hold=max(Z_hat,0.10);
end

F=[1 0 Ts 0;0 1 0 Ts;0 0 1 0;0 0 0 1];
H=[1 0 0 0;0 1 0 0]; I4=eye(4);

pose_matrix_ok=isequal(size(T_camera2base),[4 4]) && ...
all(isfinite(T_camera2base(:)));
R_base_camera=eye(3); t_base_camera=zeros(3,1); pose_ok=false;

if pose_matrix_ok
R_candidate=T_camera2base(1:3,1:3);
t_candidate=T_camera2base(1:3,4);
pose_ok=norm(R_candidate'*R_candidate-eye(3),'fro')<1e-3 && ...
abs(det(R_candidate)-1.0)<1e-3 && ...
norm(T_camera2base(4,:)-[0 0 0 1])<1e-6 && ...
all(isfinite(t_candidate));
if pose_ok, R_base_camera=R_candidate; t_base_camera=t_candidate; end
end

measurement_vectors_ok=numel(z_meas)==2 && numel(e)==2 && ...
all(isfinite(z_meas(:))) && all(isfinite(e(:)));
vision_safe=safe_valid && measurement_vectors_ok;

if ~vision_safe
time_since_visible=inf; target_tracking_active=false; e_hold=zeros(2,1);
elseif target_is_new && target_visible
time_since_visible=0.0; target_tracking_active=true; e_hold=reshape(e,2,1);
if isfinite(z) && z>1e-4, z_hold=z; end
else
time_since_visible=min(time_since_visible+Ts,target_lost_timeout+Ts);
if time_since_visible>=target_lost_timeout
target_tracking_active=false; e_hold=zeros(2,1);
end
end

measurement_available=vision_safe && target_is_new && target_visible && ...
pose_ok && isfinite(z) && z>1e-4;
z_base=zeros(2,1); R_measurement_base=R_ekf;

if measurement_available
p_target_camera=[z_meas(1);z_meas(2);z];
p_target_base=R_base_camera*p_target_camera+t_base_camera;
z_base=p_target_base(1:2);
measurement_rotation=R_base_camera(1:2,1:2);
R_measurement_base=measurement_rotation*R_ekf*measurement_rotation';
R_measurement_base=0.5*(R_measurement_base+R_measurement_base');
measurement_available=all(isfinite(z_base(:))) && ...
all(isfinite(R_measurement_base(:)));
end

if ~initialized
if measurement_available
x_hat=[z_base(1);z_base(2);0;0]; P=P0;
initialized=true; measurement_accepted=true;
end
else
x_pred=F*x_hat; P_pred=F*P*F'+Q_ekf; P_pred=0.5*(P_pred+P_pred');
x_hat=x_pred; P=P_pred;

if measurement_available
innovation=z_base-H*x_pred; S=H*P_pred*H'+R_measurement_base;
if all(isfinite(S(:))) && rcond(S)>1e-12
innovation_nis=innovation'*(S\innovation);
else
innovation_nis=inf;
end

if isfinite(innovation_nis) && innovation_nis<=gate
K=(P_pred*H')/S; x_hat=x_pred+K*innovation; A=I4-K*H;
P=A*P_pred*A'+K*R_measurement_base*K';
P=0.5*(P+P'); measurement_accepted=true;
end
end
end

if measurement_accepted
time_since_accepted=0.0;
valid_streak=min(valid_streak+1.0,required_valid_frames);
if valid_streak>=required_valid_frames, ekf_ready=true; end

else
if target_is_new && ~ekf_ready, valid_streak=0.0; end
time_since_accepted=time_since_accepted+Ts;
end

ekf_ok=all(isfinite(x_hat(:))) && all(isfinite(P(:))) && ...
all(diag(P)>=0.0) && norm(P-P','fro')<1e-6;

if time_since_accepted>=measurement_reset_timeout || ~ekf_ok
x_hat=zeros(4,1); P=P0; time_since_accepted=0.0; initialized=false;
valid_streak=0.0; ekf_ready=false; measurement_accepted=false;
end

ekf_state=x_hat; ekf_covariance=P;

if initialized && ekf_ready
v_target_hat=x_hat(3:4);
else
v_target_hat=zeros(2,1); ekf_state(3:4)=zeros(2,1);
end

ekf_initialized=initialized && ekf_ready;

if controller_enable && enable_p && vision_safe && target_tracking_active
v_p=z_hold*[Kpx*e_hold(1);Kpy*e_hold(2)];
else
v_p=zeros(2,1);
end

v_target_camera_xy=zeros(2,1);

if initialized && ekf_ready && pose_ok
v_target_base_3d=[x_hat(3);x_hat(4);0];
v_target_camera_3d=R_base_camera'*v_target_base_3d;
v_target_camera_xy=v_target_camera_3d(1:2);
end

if controller_enable && enable_ff && vision_safe && ...
initialized && ekf_ready && pose_ok
v_ff=k_ff*v_target_camera_xy;
else
v_ff=zeros(2,1);
end

v_task_raw=v_p+v_ff;

control_active=controller_enable && vision_safe && ...
((enable_p && target_tracking_active) || ...
(enable_ff && initialized && ekf_ready && pose_ok));

if control_active
filter_alpha=Ts/(task_velocity_filter_tau+Ts);
v_issued_hold=v_issued_hold+filter_alpha*(v_task_raw-v_issued_hold);
else
v_issued_hold=zeros(2,1);
end

v_issued=v_issued_hold;
camera_velocity=[v_issued;0;0;0;0];
acceleration_active=false;

controller_ok=all(isfinite(v_p(:))) && all(isfinite(v_ff(:))) && ...
all(isfinite(v_task_raw(:))) && all(isfinite(v_issued(:)));

if ~controller_ok
v_p=zeros(2,1); v_ff=zeros(2,1); v_task_raw=zeros(2,1);
v_issued_hold=zeros(2,1); v_issued=zeros(2,1);
camera_velocity=zeros(6,1); control_active=false; e_hold=zeros(2,1);
time_since_visible=inf; target_tracking_active=false;
end
end

== matlab function Copy_of_single_camera_q_dot/Redundant Visual Velocity Solver ==
  data: v_issued input; qdot_raw output; e input; z input; J_camera input; q input; safe_valid input; control_active input; controller_ok input; kinematics_valid input; solver_parameters input; q_nominal input; q_min input; q_max input; sigma_min output; damping_used output; singularity_scale output; solver_valid output
function [qdot_raw,sigma_min,damping_used,singularity_scale,solver_valid] = fcn( ...
v_issued,e,z,J_camera,q,safe_valid,control_active,controller_ok, ...
kinematics_valid,solver_parameters,q_nominal,q_min,q_max)
%#codegen
% v_issued：经过任务空间低通后的二维相机平移速度指令。
% J_camera：相机光学坐标系表达、顺序为 [vx;vy;vz;wx;wy;wz]。
% 主任务只有图像中心 2 维约束，关节求解可自然使用完整 6 维相机运动。

persistent feature_hold depth_hold
if isempty(depth_hold)
feature_hold=zeros(2,1); depth_hold=0.50;
end

qdot_raw=zeros(7,1); sigma_min=0.0; damping_used=0.0;
singularity_scale=0.0; solver_valid=false;

q=reshape(q,7,1); q_nominal=reshape(q_nominal,7,1);
q_min=reshape(q_min,7,1); q_max=reshape(q_max,7,1);

input_ok=numel(v_issued)==2 && numel(e)==2 && ...
isequal(size(J_camera),[6 7]) && numel(solver_parameters)>=9 && ...
all(isfinite(v_issued(:))) && all(isfinite(e(:))) && ...
all(isfinite(J_camera(:))) && all(isfinite(q(:))) && ...
all(isfinite(q_nominal(:))) && all(isfinite(q_min(:))) && ...
all(isfinite(q_max(:))) && all(q_max>q_min) && ...
all(isfinite(solver_parameters(1:9)));

if ~input_ok
feature_hold=zeros(2,1); depth_hold=0.50; return;
end

lambda_min=solver_parameters(1); lambda_max=solver_parameters(2);
sigma_stop=solver_parameters(3); sigma_warn=solver_parameters(4);
posture_gain=solver_parameters(5); depth_min=solver_parameters(6);
depth_max=solver_parameters(7); depth_gain=solver_parameters(8);
minimum_depth=solver_parameters(9);

parameter_ok=lambda_min>0.0 && lambda_max>=lambda_min && ...
sigma_stop>=0.0 && sigma_warn>sigma_stop && posture_gain>=0.0 && ...
depth_min>minimum_depth && depth_max>depth_min && ...
depth_gain>=0.0 && minimum_depth>0.0;

if ~parameter_ok
feature_hold=zeros(2,1); depth_hold=0.50; return;
end

if safe_valid && isfinite(z) && z>minimum_depth
feature_hold=reshape(e,2,1); depth_hold=z;
elseif ~safe_valid
feature_hold=zeros(2,1); depth_hold=max(depth_min,minimum_depth);
end

singular_values=svd(J_camera);
sigma_min=singular_values(6);

if sigma_min<=sigma_stop
singularity_scale=0.0; damping_used=lambda_max;
elseif sigma_min>=sigma_warn
singularity_scale=1.0; damping_used=lambda_min;
else
ratio=(sigma_min-sigma_stop)/(sigma_warn-sigma_stop);
singularity_scale=ratio*ratio*(3.0-2.0*ratio);
damping_used=lambda_max-(lambda_max-lambda_min)*singularity_scale;
end

solver_valid=isfinite(sigma_min) && isfinite(damping_used) && ...
isfinite(singularity_scale);

if ~solver_valid
qdot_raw=zeros(7,1); return;
end

if ~(safe_valid && control_active && controller_ok && kinematics_valid)
qdot_raw=zeros(7,1); return;
end

x=feature_hold(1); y=feature_hold(2); Z=max(depth_hold,minimum_depth);

L=[-1.0/Z 0 x/Z x*y -(1.0+x*x) y; ...
0 -1.0/Z y/Z 1.0+y*y -x*y -x];

J_image=L*J_camera;
normal_matrix=J_image*J_image'+damping_used*damping_used*eye(2);

if ~(all(isfinite(normal_matrix(:))) && rcond(normal_matrix)>1e-12)
solver_valid=false; qdot_raw=zeros(7,1); return;
end

J_image_damped=J_image'/normal_matrix;
feature_rate_command=-(reshape(v_issued,2,1)/Z);
qdot_task=J_image_damped*feature_rate_command;
N_image=eye(7)-J_image_damped*J_image;

% 简单、低参数的关节中心和软限位回避种子。
joint_range=q_max-q_min;
posture_error=(q-q_nominal)./(0.5*joint_range);
qdot_seed=-posture_gain*posture_error;
soft_zone=0.12*joint_range;

for joint_index=1:7
lower_soft=q_min(joint_index)+soft_zone(joint_index);
upper_soft=q_max(joint_index)-soft_zone(joint_index);

if q(joint_index)<lower_soft
normalized_distance=(lower_soft-q(joint_index))/soft_zone(joint_index);
qdot_seed(joint_index)=qdot_seed(joint_index)+ ...
2.0*posture_gain*normalized_distance*normalized_distance;
elseif q(joint_index)>upper_soft
normalized_distance=(q(joint_index)-upper_soft)/soft_zone(joint_index);
qdot_seed(joint_index)=qdot_seed(joint_index)- ...
2.0*posture_gain*normalized_distance*normalized_distance;
end
end

qdot_null=N_image*qdot_seed;

% 深度只在安全区之外工作，并投影到图像主任务零空间。
depth_rate_command=0.0;

if Z<depth_min
depth_rate_command=depth_gain*(depth_min-Z);
elseif Z>depth_max
depth_rate_command=-depth_gain*(Z-depth_max);
end

L_depth=[0 0 -1.0 -Z*y Z*x 0];
J_depth=L_depth*J_camera;
J_depth_null=J_depth*N_image;

depth_denominator=J_depth_null*J_depth_null'+ ...
damping_used*damping_used;

qdot_depth=zeros(7,1);

if depth_rate_command~=0.0 && ...
isfinite(depth_denominator) && depth_denominator>1e-12
qdot_depth=N_image*J_depth'*(depth_rate_command/depth_denominator);
end

% 奇异度缩放作用于主任务、零空间姿态和深度任务的总和。
% sigma_min<=sigma_stop 时三类运动均平滑降为零。
qdot_raw=singularity_scale*(qdot_task+qdot_null+qdot_depth);

solver_valid=all(isfinite(qdot_raw(:)));
if ~solver_valid, qdot_raw=zeros(7,1); end
end

== matlab function Copy_of_single_camera_q_dot/Final Joint Command Guard ==
  data: qdot_raw input; qdot_command output; q input; safe_valid input; control_active input; solver_valid input; guard_parameters input; qdot_limit input; qddot_limit input; q_min input; q_max input; velocity_scale output; acceleration_scale output; position_scale output; guard_valid output
function [qdot_command,velocity_scale,acceleration_scale,position_scale,guard_valid] = fcn( ...
qdot_raw,q,safe_valid,control_active,solver_valid,guard_parameters, ...
qdot_limit,qddot_limit,q_min,q_max)
%#codegen
% 全系统最终关节命令处理：
% 整体速度缩放 -> 逐关节软位置边界 -> 整体加速度缩放。
% 接近上限只限制正速度，接近下限只限制负速度，其他关节正常运动。
% 任务空间低通已在前级控制器中完成，本模块不再重复低通。

persistent previous_command initialized
if isempty(initialized)
previous_command=zeros(7,1); initialized=true;
end

qdot_command=zeros(7,1); velocity_scale=0.0; acceleration_scale=0.0;
position_scale=0.0; guard_valid=false;
qdot_raw=reshape(qdot_raw,7,1); q=reshape(q,7,1);
qdot_limit=reshape(qdot_limit,7,1);
qddot_limit=reshape(qddot_limit,7,1);
q_min=reshape(q_min,7,1); q_max=reshape(q_max,7,1);

input_ok=numel(guard_parameters)==2 && ...
all(isfinite(qdot_raw(:))) && all(isfinite(q(:))) && ...
all(isfinite(qdot_limit(:))) && all(qdot_limit>0.0) && ...
all(isfinite(qddot_limit(:))) && all(qddot_limit>0.0) && ...
all(isfinite(q_min(:))) && all(isfinite(q_max(:))) && ...
all(q_max>q_min) && all(isfinite(guard_parameters(1:2)));
if ~input_ok
previous_command=zeros(7,1); return;
end

Ts=guard_parameters(1); soft_margin=guard_parameters(2);
parameter_ok=Ts>0.0 && soft_margin>0.0;
if ~parameter_ok
previous_command=zeros(7,1); return;
end

target_velocity=zeros(7,1);
% 使能或数据失效时把目标速度置零，并通过加速度限制缓降。
if safe_valid && control_active && solver_valid
target_velocity=qdot_raw;
end

% 整体速度缩放：任一关节达到速度限值时，7维方向同比例保留。
maximum_velocity_ratio=max(abs(target_velocity)./qdot_limit);
velocity_scale=1.0/max(1.0,maximum_velocity_ratio);
velocity_limited=target_velocity*velocity_scale;

% 逐关节限制靠近位置边界时的向外速度，不影响返回速度和其他关节。
position_scale=1.0;
for joint_index=1:7
local_scale=1.0;

if velocity_limited(joint_index)>0.0
distance_to_limit=q_max(joint_index)-q(joint_index);
local_scale=min(max(distance_to_limit/soft_margin,0.0),1.0);
elseif velocity_limited(joint_index)<0.0
distance_to_limit=q(joint_index)-q_min(joint_index);
local_scale=min(max(distance_to_limit/soft_margin,0.0),1.0);
end

velocity_limited(joint_index)=velocity_limited(joint_index)*local_scale;
position_scale=min(position_scale,local_scale);
end

% 整体加速度缩放：限制本周期7维速度变化，保持变化方向。
delta_velocity=velocity_limited-previous_command;
maximum_acceleration_ratio=max(abs(delta_velocity)./(qddot_limit*Ts));
acceleration_scale=1.0/max(1.0,maximum_acceleration_ratio);
qdot_command=previous_command+delta_velocity*acceleration_scale;

% 到达位置边界后，只禁止对应关节继续向外，允许其返回。
for joint_index=1:7
if q(joint_index)>=q_max(joint_index) && qdot_command(joint_index)>0.0
qdot_command(joint_index)=0.0;
position_scale=0.0;
elseif q(joint_index)<=q_min(joint_index) && qdot_command(joint_index)<0.0
qdot_command(joint_index)=0.0;
position_scale=0.0;
end
end

guard_valid=all(isfinite(qdot_command(:)));
if guard_valid
previous_command=qdot_command;
else
qdot_command=zeros(7,1); previous_command=zeros(7,1);
velocity_scale=0.0; acceleration_scale=0.0; position_scale=0.0;
end
end

== matlab function Copy_of_single_camera_q_dot/Joint Velocity Publisher/Pack Seven Joint Velocities ==
  data: qdot_command input; data output; current_length output; received_length output
function [data,current_length,received_length] = fcn(qdot_command)
%#codegen
data=zeros(128,1);
data(1:7)=reshape(qdot_command,7,1);
current_length=uint32(7);
received_length=uint32(7);
end

== matlab function Copy_of_single_camera_q_dot/Target ROS2 Subscriber/Unpack ==
  data: data input; target_data output size=[4 1]; is_new input size=1; t input size=1; target_count output size=1; target_age output size=1
function [target_data,target_count,target_age] = fcn(data,is_new,t)
%#codegen
% target_data = [valid; u; v; depth_m]

persistent last_data last_count last_time

if isempty(last_count)
    last_data  = zeros(4,1);
    last_count = 0.0;
    last_time  = -1.0e6;
end

if is_new
    n = numel(data);

    last_data = zeros(4,1);

    if n >= 1, last_data(1) = data(1); end  % valid
    if n >= 2, last_data(2) = data(2); end  % u
    if n >= 3, last_data(3) = data(3); end  % v
    if n >= 4, last_data(4) = data(4); end  % depth_m

    last_count = double(n);
    last_time  = t;
end

target_data  = last_data;
target_count = last_count;
target_age   = max(0.0,t-last_time);
end

== matlab function Copy_of_single_camera_q_dot/Kinematics Feedback/MATLAB Function ==
  data: J_camera_base_wv input; camera_twist_measured output; qdot_measured input; T_camera2base input; joint_count input; joint_age input; feedback_timeout input; kinematics_valid output; T_camera2base_out output; J_camera output
function [camera_twist_measured,kinematics_valid,T_camera2base_out,J_camera] = fcn( ...
    J_camera_base_wv,qdot_measured,T_camera2base,joint_count,joint_age,feedback_timeout)
%#codegen
% Get Jacobian 输出为 Base 表达的 [omega;v]。
% 本函数输出相机光学坐标系表达的 [v;omega] 和完整 6x7 Jacobian。

camera_twist_measured = zeros(6,1);
kinematics_valid = false;
T_camera2base_out = eye(4);
J_camera = zeros(6,7);
qdot_measured = reshape(qdot_measured,7,1);

input_ok = joint_count >= 7 && isfinite(joint_age) && ...
    isfinite(feedback_timeout) && feedback_timeout > 0.0 && ...
    joint_age >= 0.0 && joint_age <= feedback_timeout && ...
    all(isfinite(qdot_measured(:))) && ...
    isequal(size(J_camera_base_wv),[6 7]) && ...
    all(isfinite(J_camera_base_wv(:))) && ...
    isequal(size(T_camera2base),[4 4]) && ...
    all(isfinite(T_camera2base(:)));

if ~input_ok
    return;
end

R_base_camera = T_camera2base(1:3,1:3);
pose_ok = norm(R_base_camera'*R_base_camera-eye(3),'fro') < 1e-3 && ...
    abs(det(R_base_camera)-1.0) < 1e-3 && ...
    norm(T_camera2base(4,:)-[0 0 0 1]) < 1e-6;
if ~pose_ok
    return;
end

% 先把 [omega;v] 改成统一的 [v;omega]。
J_base_vw = J_camera_base_wv([4 5 6 1 2 3],:);
R_camera_base = R_base_camera';
rotation6 = [R_camera_base zeros(3);zeros(3) R_camera_base];

% Jacobian 已经是在 camera_link 原点计算，因此这里只改变表达坐标系，
% 不再重复加入相机安装平移偏置。
J_camera = rotation6*J_base_vw;
camera_twist_measured = J_camera*qdot_measured;
T_camera2base_out = T_camera2base;

kinematics_valid = all(isfinite(J_camera(:))) && ...
    all(isfinite(camera_twist_measured(:)));
if ~kinematics_valid
    J_camera = zeros(6,7);
    camera_twist_measured = zeros(6,1);
end
end
